simulink model "tractor_mu1109"  (R2022b)
settings: Solver=FixedStepDiscrete  StartTime=0.0  StopTime=20  FixedStep=0.001  RelTol=1e-3
model workspace (MAT data in the model file):
  P : object (value not decoded)
  w_2 : Simulink.Parameter (value not decoded)
undefined symbols (not defined in the file): A, a, B, b, C, D, DiscIntNeverNeededParam, Iz, K, k1, K1, k2, K2, L1, L2, m, magnitude, Phi, Sample_time, Steer_Ratio
libraries: simulink x26, slpidlib x13, Solver_SF x1, dsparch4 x1
(part 3 of 7)

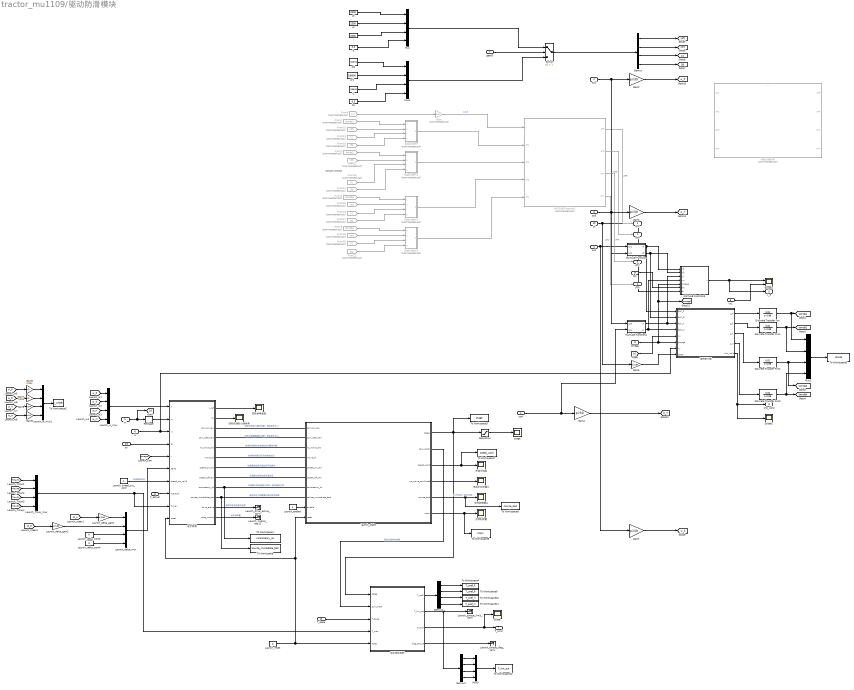
== system tractor_mu1109/驱动防滑模块 ==
  note: 300000
      | 450000
  sp1 : Inport
  sp2 : Inport  Port=2
  sp3 : Inport  Port=3
  sp4 : Inport  Port=4
  vx : Inport  Port=5
  vy : Inport  Port=6
  gearD : Inport  Port=7
  omega : Inport  Port=8
  brk : Inport  Port=9
  st : Inport  Port=10
  T_base : Inport  Port=11
  T_actual : Inport  Port=12
  ax : Inport  Port=13
  Demux : Demux
  Demux1 : Demux
  Demux2 : Demux
  Discrete Transfer Fcn{,1..3} (4 alike) : DiscreteTransferFcn  Numerator=[0.02]  Denominator=[1 -0.98]
  From10 : From  Commented=on  GotoTag=pf
  From{11,13,16,20} (4 alike) : From  Commented=on  GotoTag=i
  From12 : From  Commented=on  GotoTag=pf
  From{14,17..18,21} (4 alike) : From  Commented=on  GotoTag=b
  From15 : From  Commented=on  GotoTag=pr
  From19 : From  Commented=on  GotoTag=pr
  From2 : From  Commented=on  GotoTag=lamda1  TagVisibility=global
  From3 : From  Commented=on  GotoTag=lamda2  TagVisibility=global
  From4 : From  Commented=on  GotoTag=lamda3  TagVisibility=global
  From5 : From  Commented=on  GotoTag=lamda4  TagVisibility=global
  From6 : From  Commented=on  GotoTag=v
  Gain : Gain  Commented=on  Gain=3.6
  Gain{1..4} (4 alike) : Gain  Gain=pi/30
  Gain5 : Gain  Gain=pi/180
  Gain6 : Gain  Gain=0.834
  Gain7 : Gain  Gain=0.834
  Gain8 : Gain  Gain=0.94
  Gain9 : Gain  Gain=0.94
  Launch_Tmax_mux : Mux
  Launch_delta_gain1 : Gain  Gain=pi/180
  Launch_delta_gain2 : Gain  Gain=pi/180
  Launch_delta_mux : Mux
  Launch_delta_zero3 : Constant  Value=0
  Launch_delta_zero4 : Constant  Value=0
  Launch_drive_active_term : Terminator
  Launch_enable : Constant
  Launch_motion_obs12 : Terminator
  Launch_reset : Constant  Value=0
  Launch_speed_src_valid : Constant
  Launch_torque_diag_term : Terminator
  Launch_torque_limit_term : Terminator
  Launch_w_mux : Mux
  Launch_w_mux1 : Mux
  MATLAB Function : MATLAB Function  TreatAsAtomicUnit=on
  MATLAB Function1 : MATLAB Function  TreatAsAtomicUnit=on
  MATLAB Function2 : MATLAB Function  Commented=on  TreatAsAtomicUnit=on
  MATLAB Function3 : MATLAB Function  TreatAsAtomicUnit=on
  Mux{,1..3} (4 alike) : Mux
  Reshape : Reshape  OutputDimensionality=Customize  OutputDimensions=[1 1]
  Saturation : Saturate  UpperLimit=10  LowerLimit=0
  Scope : Scope
  Scope1 : Scope  NumInputPorts=2
  Scope2 : Scope
  Subsystem : Subsystem  Commented=on
  Subsystem1 : Subsystem  Commented=on
  Subsystem2 : Subsystem  Commented=on
  Subsystem3 : Subsystem  Commented=on
  Switch : Switch  Criteria=u2 > Threshold  Threshold=1  SaturateOnIntegerOverflow=off  InputSameDT=off
  To Workspace : ToWorkspace  VariableName=source_immediate_bad  SampleTime=-1
  To Workspace1 : ToWorkspace  VariableName=consistency_ok  SampleTime=-1
  To Workspace10 : ToWorkspace  VariableName=T_pref_rl  SampleTime=-1
      settings: Save2DSignal=2-D array (concatenate along first dimension)
  To Workspace11 : ToWorkspace  VariableName=T_pref_rr  SampleTime=-1
      settings: Save2DSignal=2-D array (concatenate along first dimension)
  To Workspace12 : ToWorkspace  VariableName=T_lim_out  SampleTime=-1
  To Workspace2 : ToWorkspace  VariableName=v_wheel  SampleTime=-1
  To Workspace3 : ToWorkspace  VariableName=stage  SampleTime=-1
  To Workspace4 : ToWorkspace  VariableName=T_pref_fl  SampleTime=-1
      settings: Save2DSignal=2-D array (concatenate along first dimension)
  To Workspace5 : ToWorkspace  VariableName=lamda  SampleTime=-1
  To Workspace6 : ToWorkspace  VariableName=nspin  SampleTime=-1
  To Workspace7 : ToWorkspace  VariableName=speed_valid  SampleTime=-1
  To Workspace8 : ToWorkspace  VariableName=source_bad  SampleTime=-1
  To Workspace9 : ToWorkspace  VariableName=T_pref_fr  SampleTime=-1
      settings: Save2DSignal=2-D array (concatenate along first dimension)
  b : Constant  Value=0.3
  b1 : Constant  Value=0.3
  i : Constant  Value=2000
  i1 : Constant  Value=35000
  launch_state : Stateflow chart  TreatAsAtomicUnit=on
  pf : Constant  Value=2000
  pf1 : Constant  Value=90000
  pr : Constant  Value=2500
  pr1 : Constant  Value=105000
  stage : Scope
  vx1 : InportShadow  Port=5
  信号故障确认 : Scope
  四轮参考速度 : Scope
  四轮轮端轮心速度差 : Scope
  未起步状态确认 : Scope
  滑转率计算 : Subsystem
  空转轮数量 : Scope
  起步扭矩控制 : MATLAB Function  TreatAsAtomicUnit=on
  起步探测 : MATLAB Function  TreatAsAtomicUnit=on
  车速可信度 : Scope
  转矩协调控制 : Stateflow chart  Commented=on  TreatAsAtomicUnit=on
      settings: PortSchema="{\"entries\":[{\"content\":{\"sides\":[{\"content\":{\"connectorIds\":[\"In2\",\"In3\",\"In4\",\"In5\"]},\"type\":\"ConnectorPlacement.EquallySpacedRectSide\",\"uuid\":\"973a9b84-73ad-47b8-a26a-d7aec675acf5\"},{\"content\":{\"connectorIds\":[\"Out1\",\"Out2\",\"Out3\",\"Out4\"],\"side\":\"RIGHT\"},\"type\":\"ConnectorPlacement.EquallySpacedRectSide\",\"uuid\":\"de1e0d9b-25bd-4ac7-be2f-c0268a60ba4f\"},{\"content\":{\"connectorIds\":[\"In1\"],\"side\":\"TOP\"},\"type\":\"ConnectorPlacement.EquallySpacedRectSide\",\"uuid\":\"9ce864d3-2ff1-442a-967b-03df7267dcea\"}]},\"type\":\"ConnectorPlacement.EquallySpacedConnector\",\"uuid\":\"50a94803-c5b1-4606-ba3c-9c5c7d907f69\"}],\"packageUris\":[\"http://schema.mathworks.com/mf0/Connector/R2020b\"],\"version\":\"1.0\"}"
  dTfl : Outport
  dTfr : Outport  Port=2
  dTrl : Outport  Port=3
  dTrr : Outport  Port=4
  v_e : Outport  Port=5
  slip_valid : Outport  Port=6
  T_cmd : Outport  Port=7
  tag scope: lamda1=global, lamda2=global, lamda3=global, lamda4=global, w_fl=global, w_fr=global, w_rl=global, w_rr=global
  wires:
  [w_fl] -> Launch_w_mux/1
  pf/1 -> Mux/1
  pr/1 -> Mux/2
  i/1 -> Mux/3
  [st_R] -> Launch_delta_gain2/1
  b/1 -> Mux/4
  [TMaxRL] -> Launch_Tmax_mux/3
  pf1/1 -> Mux1/1
  pr1/1 -> Mux1/2
  Mux1/1 -> Switch/3
  Subsystem/1(dT1) -> MATLAB Function2/2(dT1)
  i1/1 -> Mux1/3
  b1/1 -> Mux1/4
  launch_state/6(nspin) -> To Workspace6/1, 空转轮数量/1
  From6/1 -> Gain/1
  From2/1 -> Subsystem/1(lamda1)
  From10/1 -> Subsystem/2(p)
  Subsystem3/1(dT1) -> MATLAB Function2/5(dT4)
  From11/1 -> Subsystem/3(i)
  [w_fr] -> Launch_w_mux/2
  From18/1 -> Subsystem/4(b)
  Launch_Tmax_mux/1 -> 起步探测/9(T_max), 起步扭矩控制/4(T_max)
  From4/1 -> Subsystem2/1(lamda3)
  From3/1 -> Subsystem1/1(lamda2)
  From12/1 -> Subsystem1/2(p)
  From14/1 -> Subsystem1/4(b)
  From13/1 -> Subsystem1/3(i)
  sp1/1 -> MATLAB Function/1(sp1), Gain1/1
  From15/1 -> Subsystem2/2(p)
  MATLAB Function2/4(dTrr) -> dTrr/1  "dTrr"
  From16/1 -> Subsystem2/3(i)
  起步扭矩控制/2(T_lim_out) -> Demux2/1, Launch_torque_limit_term/1
  Launch_enable/1 -> launch_state/9(enable)
  From17/1 -> Subsystem2/4(b)
  From5/1 -> Subsystem3/1(lamda4)
  From21/1 -> Subsystem3/4(b)
  From19/1 -> Subsystem3/2(p)
  [st_L] -> Launch_delta_gain1/1
  From20/1 -> Subsystem3/3(i)
  Launch_reset/1 -> 起步扭矩控制/5(reset), launch_state/10(reset), 起步探测/10(reset)
  [TMaxFL] -> Launch_Tmax_mux/1
  st/1 -> MATLAB Function3/7(st), Gain5/1
  [TMaxFR] -> Launch_Tmax_mux/2
  [TMaxRR] -> Launch_Tmax_mux/4
  Mux/1 -> Switch/1
  gearD/1 -> Switch/2
  MATLAB Function2/1(dTfl) -> dTfl/1  "dTfl"
  Launch_w_mux/1 -> 起步探测/1(w)
  launch_state/1(stage) -> To Workspace3/1, Saturation/1, 起步扭矩控制/1(stage)  "工作状态（起步过程）"
  Gain/1 -> MATLAB Function2/1(v)  "km/h"
  Subsystem1/1(dT1) -> MATLAB Function2/3(dT2)
  [w_rl] -> Launch_w_mux/3
  launch_state/2(spin_mask) -> 起步扭矩控制/2(spin_mask)  "四轮空转锁存结果"
  Subsystem2/1(dT1) -> MATLAB Function2/4(dT3)
  launch_state/3(speed_valid) -> To Workspace7/1, 车速可信度/1
  launch_state/4(no_move_confirmed) -> 未起步状态确认/1
  launch_state/5(source_bad) -> To Workspace8/1, 信号故障确认/1
  T_base/1 -> 起步扭矩控制/3(T_base)
  Switch/1 -> Demux/1
  sp2/1 -> MATLAB Function/2(sp2), Gain2/1
  MATLAB Function2/2(dTfr) -> dTfr/1  "dTfr"
  MATLAB Function2/3(dTrl) -> dTrl/1  "dTrl"
  ax/1 -> 起步探测/4(ax)
  sp3/1 -> MATLAB Function1/1(sp3), Gain3/1
  Gain2/1 -> [w_fr]
  起步扭矩控制/3(T_cmd) -> Scope/1, T_cmd/1
  起步扭矩控制/4(diag_torque) -> Launch_torque_diag_term/1
  sp4/1 -> MATLAB Function1/2(sp4), Gain4/1
  [w_rr] -> Launch_w_mux/4
  Launch_delta_gain1/1 -> Launch_delta_mux/1
  Launch_delta_gain2/1 -> Launch_delta_mux/2
  Launch_delta_zero3/1 -> Launch_delta_mux/3
  Launch_delta_zero4/1 -> Launch_delta_mux/4
  Demux/1 -> [pf]
  Demux/2 -> [pr]
  滑转率计算/4(s_rr) -> Discrete Transfer Fcn3/1
  Demux/3 -> [i]
  Demux/4 -> [b]
  Gain3/1 -> [w_rl]
  MATLAB Function/1(vfl) -> MATLAB Function3/1(vfl), 滑转率计算/1(Roll_fl)
  MATLAB Function/2(vfr) -> MATLAB Function3/2(vfr), 滑转率计算/2(Roll_fr)
  brk/1 -> MATLAB Function3/6(brk)
  MATLAB Function1/1(vrl) -> MATLAB Function3/3(vrl), 滑转率计算/3(Roll_rl)
  MATLAB Function1/2(vrr) -> MATLAB Function3/4(vrr), 滑转率计算/4(Roll_rr)
  omega/1 -> [omega], MATLAB Function3/5(omega), 滑转率计算/6(omega)
  [v] -> 滑转率计算/5(vx)
  Gain5/1 -> 滑转率计算/8(derta)
  vy/1 -> 滑转率计算/7(vy), 起步探测/3(vy)
  vx/1 -> [v], Reshape/1
  Gain1/1 -> [w_fl]
  [omega] -> 起步探测/5(r)
  Launch_delta_mux/1 -> 起步探测/6(delta)
  Launch_speed_src_valid/1 -> 起步探测/7(speed_src_valid)  "车速源有效性"
  Gain4/1 -> [w_rr]
  MATLAB Function3/1(v) -> Scope1/1, v_e/1
  vx1/1 -> Scope1/2
  滑转率计算/1(s_fl) -> Discrete Transfer Fcn/1
  滑转率计算/2(s_fr) -> Discrete Transfer Fcn1/1
  滑转率计算/3(s_rl) -> Discrete Transfer Fcn2/1
  滑转率计算/5(slip_valid) -> slip_valid/1, Scope2/1
  起步探测/1(v_ref) -> 四轮参考速度/1
  起步探测/2(dv) -> 四轮轮端轮心速度差/1
  起步探测/3(spin_on_raw) -> launch_state/1(spin_on_raw)  "四轮空转进入瞬时判据，满足条件为 1"
  起步探测/4(spin_clear_raw) -> launch_state/2(spin_clear_raw)  "四轮空转解除瞬时判据，满足条件为 1"
  起步探测/5(no_move_raw) -> launch_state/3(no_move_raw)  "检测到车辆仍未有效起步的瞬时判据"
  起步探测/6(move_ok) -> launch_state/4(move_ok)  "检测到车辆已经开始有效运动"
  起步探测/7(speed_on_raw) -> launch_state/5(speed_on_raw)  "车速源有效且车速达到可信条件"
  起步探测/8(speed_off_raw) -> launch_state/6(speed_off_raw)  "车速源立即失效或车速过低"
  起步探测/9(consistency_ok) -> To Workspace1/1, launch_state/7(consistency_ok)  "车速微分和加速度之间的一致性是否正常"
  起步探测/10(source_immediate_bad) -> To Workspace/1, launch_state/8(source_immediate_bad)  "是否存在立即需要处理的信号故障"
  起步探测/11(drive_active) -> Launch_drive_active_term/1  "是否存在有效驱动扭矩"
  起步探测/12(diag_motion) -> Launch_motion_obs12/1  "运动诊断量"
  Discrete Transfer Fcn/1 -> Mux2/1, [lamda1]
  Discrete Transfer Fcn1/1 -> Mux2/2, [lamda2]
  Discrete Transfer Fcn2/1 -> Mux2/3, [lamda3]
  Discrete Transfer Fcn3/1 -> Mux2/4, [lamda4]
  Reshape/1 -> 起步探测/2(vx)
  Saturation/1 -> stage/1
  T_actual/1 -> 起步探测/8(T_actual)
  [w_fl] -> Gain6/1
  [w_fr] -> Gain7/1
  [w_rl] -> Gain8/1
  [w_rr] -> Gain9/1
  Gain6/1 -> Launch_w_mux1/1
  Gain7/1 -> Launch_w_mux1/2
  Gain8/1 -> Launch_w_mux1/3
  Gain9/1 -> Launch_w_mux1/4
  Launch_w_mux1/1 -> To Workspace2/1
  Mux2/1 -> To Workspace5/1
  起步扭矩控制/1(T_pref) -> Demux1/1
  Demux1/1 -> To Workspace4/1
  Demux1/2 -> To Workspace9/1
  Demux1/3 -> To Workspace10/1
  Demux1/4 -> To Workspace11/1
  Demux2/1 -> Mux3/1
  Demux2/2 -> Mux3/2
  Demux2/3 -> Mux3/3
  Demux2/4 -> Mux3/4
  Mux3/1 -> To Workspace12/1

== system tractor_mu1109/Dugoff轮胎模型/alpha_lamda ==
  vx : Inport
  vy : Inport  Port=2
  wz : Inport  Port=3
  delta_fl : Inport  Port=4
  delta_fr : Inport  Port=5
  w_fl : Inport  Port=6
  w_fr : Inport  Port=7
  w_rl : Inport  Port=8
  w_rr : Inport  Port=9
  Scope : Scope  NumInputPorts=4
  alpha : Subsystem
  lamda : Subsystem
  lamda_fl : Outport
  lamda_fr : Outport  Port=2
  lamda_rl : Outport  Port=3
  lamda_rr : Outport  Port=4
  alpha_fl : Outport  Port=5
  alpha_fr : Outport  Port=6
  alpha_rl : Outport  Port=7
  alpha_rr : Outport  Port=8
  wires:
  lamda/3(lamda_rl) -> Scope/3, lamda_rl/1
  lamda/4(lamda_rr) -> Scope/4, lamda_rr/1
  lamda/2(lamda_fr) -> Scope/2, lamda_fr/1
  lamda/1(lamda_fl) -> Scope/1, lamda_fl/1
  w_rr/1 -> lamda/9(w_rr)
  w_rl/1 -> lamda/8(w_rl)
  w_fr/1 -> lamda/7(w_fr)
  w_fl/1 -> lamda/6(w_fl)
  delta_fr/1 -> alpha/5(delta_fr), lamda/5(delta_fr)
  delta_fl/1 -> alpha/4(delta_fl), lamda/4(delta_fl)
  wz/1 -> alpha/3(wz), lamda/3(wz)
  vy/1 -> alpha/2(vy), lamda/2(vy)
  vx/1 -> alpha/1(vx), lamda/1(vx)
  alpha/4(alpha_rr) -> alpha_rr/1
  alpha/3(alpha_rl) -> alpha_rl/1
  alpha/2(alpha_fr) -> alpha_fr/1
  alpha/1(alpha_fl) -> alpha_fl/1

== system tractor_mu1109/Dugoff轮胎模型/pac2002 ==
  lamda_fl : Inport
  lamda_fr : Inport  Port=2
  lamda_rl : Inport  Port=3
  lamda_rr : Inport  Port=4
  alpha_fl : Inport  Port=5
  alpha_fr : Inport  Port=6
  alpha_rl : Inport  Port=7
  alpha_rr : Inport  Port=8
  Fz_fl : Inport  Port=9
  Fz_rl : Inport  Port=10
  Fz_fr : Inport  Port=11
  Fz_rr : Inport  Port=12
  mu : Inport  Port=13
  Demux : Demux
  Gain{8..11} (4 alike) : Gain  Gain=-1
  fl_dugoff : MATLAB Function  TreatAsAtomicUnit=on
  fr_dugoff : MATLAB Function  TreatAsAtomicUnit=on
  rl_dugoff : MATLAB Function  TreatAsAtomicUnit=on
  rr_dugoff : MATLAB Function  TreatAsAtomicUnit=on
  Fx_fl : Outport
  Fx_fr : Outport  Port=2
  Fx_rl : Outport  Port=3
  Fx_rr : Outport  Port=4
  Fy_fl : Outport  Port=5
  Fy_fr : Outport  Port=6
  Fy_rl : Outport  Port=7
  Fy_rr : Outport  Port=8
  wires:
  alpha_fl/1 -> fl_dugoff/4(alpha)
  Fz_fl/1 -> fl_dugoff/1(Fz)
  alpha_rr/1 -> rr_dugoff/4(alpha)
  Fz_rr/1 -> rr_dugoff/1(Fz)
  [u_fl] -> fl_dugoff/2(u)
  [u_fr] -> fr_dugoff/2(u)
  alpha_fr/1 -> fr_dugoff/4(alpha)
  [u_rl] -> rl_dugoff/2(u)
  [u_rr] -> rr_dugoff/2(u)
  lamda_fr/1 -> Gain11/1
  lamda_rl/1 -> Gain8/1
  lamda_rr/1 -> Gain9/1
  lamda_fl/1 -> Gain10/1
  alpha_rl/1 -> rl_dugoff/4(alpha)
  Gain8/1 -> rl_dugoff/3(lamda)
  Gain9/1 -> rr_dugoff/3(lamda)
  Gain10/1 -> fl_dugoff/3(lamda)
  Gain11/1 -> fr_dugoff/3(lamda)
  mu/1 -> Demux/1
  Demux/1 -> [u_fl]
  Demux/2 -> [u_fr]
  Demux/3 -> [u_rl]
  Demux/4 -> [u_rr]
  Fz_rl/1 -> rl_dugoff/1(Fz)
  Fz_fr/1 -> fr_dugoff/1(Fz)
  fl_dugoff/4(Fy) -> Fy_fl/1
  fl_dugoff/3(Fx) -> Fx_fl/1
  fr_dugoff/4(Fy) -> Fy_fr/1
  fr_dugoff/3(Fx) -> Fx_fr/1
  rl_dugoff/4(Fy) -> Fy_rl/1
  rl_dugoff/3(Fx) -> Fx_rl/1
  rr_dugoff/4(Fy) -> Fy_rr/1
  rr_dugoff/3(Fx) -> Fx_rr/1

== system tractor_mu1109/PID_Controller//直线循迹/Enabled Subsystem ==
  note: DOB:仿真步长Ts=0.001，时间常数Tao=0.1
      | 如需部署到实车需要根据实车采样频率调整
  yaw_ref : Inport
  yaw : Inport  Port=2
  beta : Inport  Port=3
  omega : Inport  Port=4
  Enable : EnablePort  StatesWhenEnabling=reset
  5500/3000 : slpidlib/PID Controller  Controller=PID  Form=Parallel  TimeDomain=Discrete-time  UseExternalTs=off  SampleTime=-1  IntegratorMethod=Forward Euler  FilterMethod=Forward Euler  ControllerParametersSource=internal  P=5500  I=3500  UseKiTs=off  D=0  N=100  UseFilter=on  TunerSelectOption=Transfer Function Based (PID Tuner App)  InitialConditionSource=internal  InitialConditionForIntegrator=0  InitialConditionForFilter=0  DifferentiatorICPrevScaledInput=0  ExternalReset=none  TrackingMode=off  Kt=1  LimitOutput=off  SatLimitsSource=internal  UpperSaturationLimit=inf  LowerSaturationLimit=-inf  LinearizeAsGain=on  AntiWindupMode=none  Kb=1  LimitIntegrator=off  UpperIntegratorSaturationLimit=inf  LowerIntegratorSaturationLimit=-inf  POutMin=[]  POutMax=[]  IOutMin=[]  IOutMax=[]  DOutMin=[]  DOutMax=[]  NOutMin=[]  NOutMax=[]  SumOutMin=[]  SumOutMax=[]  SaturationOutMin=[]  SaturationOutMax=[]  PParamMin=[]  PParamMax=[]  IParamMin=[]  IParamMax=[]  DParamMin=[]  DParamMax=[]  NParamMin=[]  NParamMax=[]  KbParamMin=[]  KbParamMax=[]  KtParamMin=[]  KtParamMax=[]  KbOutMin=[]  KbOutMax=[]  KtOutMin=[]  KtOutMax=[]  IntegratorOutMin=[]  IntegratorOutMax=[]  FilterOutMin=[]  FilterOutMax=[]  SumI1OutMin=[]  SumI1OutMax=[]  SumI2OutMin=[]  SumI2OutMax=[]  SumI3OutMin=[]  SumI3OutMax=[]  SumI4OutMin=[]  SumI4OutMax=[]  SumDOutMin=[]  SumDOutMax=[]  DifferentiatorOutMin=[]  DifferentiatorOutMax=[]  FilterDiffOutCoefMin=[]  FilterDiffOutCoefMax=[]  ReciprocalOutMin=[]  ReciprocalOutMax=[]  SumDenOutMin=[]  SumDenOutMax=[]  SumNumOutMin=[]  SumNumOutMax=[]  DivideOutMin=[]  DivideOutMax=[]  UdiffTsProdOutMin=[]  UdiffTsProdOutMax=[]  NTsProdOutMin=[]  NTsProdOutMax=[]  UintegralTsProdOutMin=[]  UintegralTsProdOutMax=[]  UngainTsProdOutMin=[]  UngainTsProdOutMax=[]  ClampingZeroOutDataTypeStr=Inherit: Inherit via back propagation  ClampingZeroOutMin=[]  ClampingZeroOutMax=[]  FilterDenConstantOutDataTypeStr=Inherit: Inherit via back propagation  FilterDenConstantOutMin=[]  FilterDenConstantOutMax=[]  PCopyOutDataTypeStr=Inherit: Inherit via back propagation  PCopyOutMin=[]  PCopyOutMax=[]  NCopyOutDataTypeStr=Inherit: Inherit via back propagation  NCopyOutMin=[]  NCopyOutMax=[]  IntegratorContinuousStateAttributes=''  IntegratorStateMustResolveToSignalObject=off  IntegratorRTWStateStorageClass=Auto  FilterContinuousStateAttributes=''  FilterStateMustResolveToSignalObject=off  FilterRTWStateStorageClass=Auto  ParallelPVariant=InternalParameters  IdealPVariant=Disabled  IVariant=InternalParameters  DVariant=InternalParameters  IntegratorVariant=Discrete  SatVariant=Disabled  AWVariant=Passthrough  PCopyVariant=Disabled  TRVariant=Disabled  FdbkBlocksVariant=Forward  IdealPFdbkVariant=Disabled  SatFdbkVariant=Disabled  DerivativeFilterVariant=ForwardEulerFilter  NVariant=InternalParameters  NCopyVariant=Disabled  FilterICVariant=InternalICsFilter  IntegratorICVariant=InternalICs  ExternalResetVariant=Disabled  TRSumVariant=Passthrough  SumFdbkVariant=Disabled  SumVariant=Sum_PID  TsampFilterVariant=InternalTs  TsampNgainVariant=Passthrough  TsampIntegralVariant=Passthrough  ExternalSaturationOutDataTypeStr=Inherit: Same as second input
  Add : Sum  Inputs=+++
  Data Type Conversion : DataTypeConversion  OutDataTypeStr=single  SaturateOnIntegerOverflow=off  RndMeth=Floor
  Data Type Conversion1 : DataTypeConversion  OutDataTypeStr=single  SaturateOnIntegerOverflow=off  RndMeth=Floor
  Discrete Transfer Fcn : DiscreteTransferFcn  Numerator=[1-exp(-0.2)]  Denominator=[1 -exp(-0.2)]
  Gain : Gain  Gain=-1
  Gain1 : Gain  Gain=-K(1)
  Gain2 : Gain  Gain=-K(2)
  Gain3 : Gain  Gain=-K(3)
  Gain4 : Gain  Gain=3
  Gain5 : Gain  Gain=0.5
  Gain6 : Gain  Gain=180/pi
  Izr_dot : simulink/Discrete/Discrete Derivative  gainval=67536  ICPrevScaledInput=0.0  OutMin=[]  OutMax=[]  OutDataType=fixdt(1, 16)  OutScaling=2^-10  DoSatur=off
  Manual Switch : ManualSwitch
  Manual Switch1 : ManualSwitch
  Subtract : Sum  Inputs=+-
  Sum : Sum  Inputs=|+-
  Sum2 : Sum  Inputs=|+-
  Mz : Outport
  wires:
  5500/3000/1 -> Data Type Conversion1/1
  yaw_ref/1 -> Sum/1
  yaw/1 -> Sum/2
  Sum/1 -> Gain/1, Gain6/1
  Sum2/1 -> Manual Switch/2
  Discrete Transfer Fcn/1 -> Gain5/1
  Subtract/1 -> Discrete Transfer Fcn/1
  Gain3/1 -> Add/3  "eyaw"
  Gain1/1 -> Add/1  "beta"
  Izr_dot/1 -> Subtract/1
  omega/1 -> Izr_dot/1, Gain2/1
  Gain2/1 -> Add/2  "omega"
  Add/1 -> Gain4/1
  beta/1 -> Gain1/1
  Gain/1 -> Gain3/1
  Manual Switch/1 -> Manual Switch1/2
  Manual Switch1/1 -> Mz/1
  Gain4/1 -> Subtract/2, Manual Switch/1, Sum2/1
  Data Type Conversion/1 -> Sum2/2  "Mz_DOB"
  Data Type Conversion1/1 -> Manual Switch1/1  "Mz_pid"
  Gain5/1 -> Data Type Conversion/1
  Gain6/1 -> 5500/3000/1

== system tractor_mu1109/PID_Controller//直线循迹/目标航向角计算 ==
  reset : Inport
  yaw : Inport  Port=2
  omega : Inport  Port=3
  Enable : EnablePort  StatesWhenEnabling=reset
  Abs : Abs  SaturateOnIntegerOverflow=off
  Add : Sum
  Constant : Constant
  Constant1 : Constant  Value=0.001
  Discrete-Time Integrator : DiscreteIntegrator  ExternalReset=rising  SampleTime=-1  ICPrevOutput=DiscIntNeverNeededParam  ICPrevScaledInput=DiscIntNeverNeededParam
  Discrete-Time Integrator1 : DiscreteIntegrator  ExternalReset=rising  SampleTime=-1  ICPrevOutput=DiscIntNeverNeededParam  ICPrevScaledInput=DiscIntNeverNeededParam
  Divide : Product  Inputs=*/
  Divide1 : Product  Inputs=*/
  Product : Product
  Saturation : Saturate  UpperLimit=999999  LowerLimit=0.1
  yaw_r : Outport
  wires:
  Constant/1 -> Divide/1
  omega/1 -> Abs/1
  Abs/1 -> Add/1
  Constant1/1 -> Add/2
  Add/1 -> Divide/2
  Divide/1 -> Discrete-Time Integrator1/1, Product/2
  yaw/1 -> Product/1
  Product/1 -> Discrete-Time Integrator/1
  Discrete-Time Integrator/1 -> Divide1/1
  Discrete-Time Integrator1/1 -> Saturation/1
  Divide1/1 -> yaw_r/1
  Saturation/1 -> Divide1/2
  reset/1 -> Discrete-Time Integrator1/2, Discrete-Time Integrator/2

== system tractor_mu1109/协同博弈扭矩分配/Subsystem ==
  Tflref : Inport
  Tfrref : Inport  Port=2
  Trlref : Inport  Port=3
  Trrref : Inport  Port=4
  Tflbase : Inport  Port=5
  Tfrbase : Inport  Port=6
  Trlbase : Inport  Port=7
  Trrbase : Inport  Port=8
  alpha : Inport  Port=9
  Constant{,1..3} (4 alike) : Constant
  Product{,1..7} (8 alike) : Product
  Sum{,2,4,6} (4 alike) : Sum  Inputs=|+-
  Sum{1,3,5,7} (4 alike) : Sum  Inputs=|++
  alpha1 : InportShadow  Port=9
  alpha2 : InportShadow  Port=9
  alpha3 : InportShadow  Port=9
  Tfl_sh : Outport
  Tfr_sh : Outport  Port=2
  Trl_sh : Outport  Port=3
  Trr_sh : Outport  Port=4
  wires:
  Tflbase/1 -> Product/1
  Constant/1 -> Sum/1
  alpha/1 -> Sum/2, Product1/2
  Sum/1 -> Product/2
  Product/1 -> Sum1/1
  Product1/1 -> Sum1/2
  Tflref/1 -> Product1/1
  Sum1/1 -> Tfl_sh/1
  Sum3/1 -> Tfr_sh/1
  Tfrref/1 -> Product3/1
  Product3/1 -> Sum3/2
  Product2/1 -> Sum3/1
  Sum2/1 -> Product2/2
  alpha1/1 -> Product3/2, Sum2/2
  Constant1/1 -> Sum2/1
  Tfrbase/1 -> Product2/1
  Trlbase/1 -> Product4/1
  Constant2/1 -> Sum4/1
  alpha2/1 -> Sum4/2, Product5/2
  Sum4/1 -> Product4/2
  Product4/1 -> Sum5/1
  Product5/1 -> Sum5/2
  Trlref/1 -> Product5/1
  Sum5/1 -> Trl_sh/1
  Sum7/1 -> Trr_sh/1
  Trrref/1 -> Product7/1
  Product7/1 -> Sum7/2
  Product6/1 -> Sum7/1
  Sum6/1 -> Product6/2
  alpha3/1 -> Product7/2, Sum6/2
  Constant3/1 -> Sum6/1
  Trrbase/1 -> Product6/1

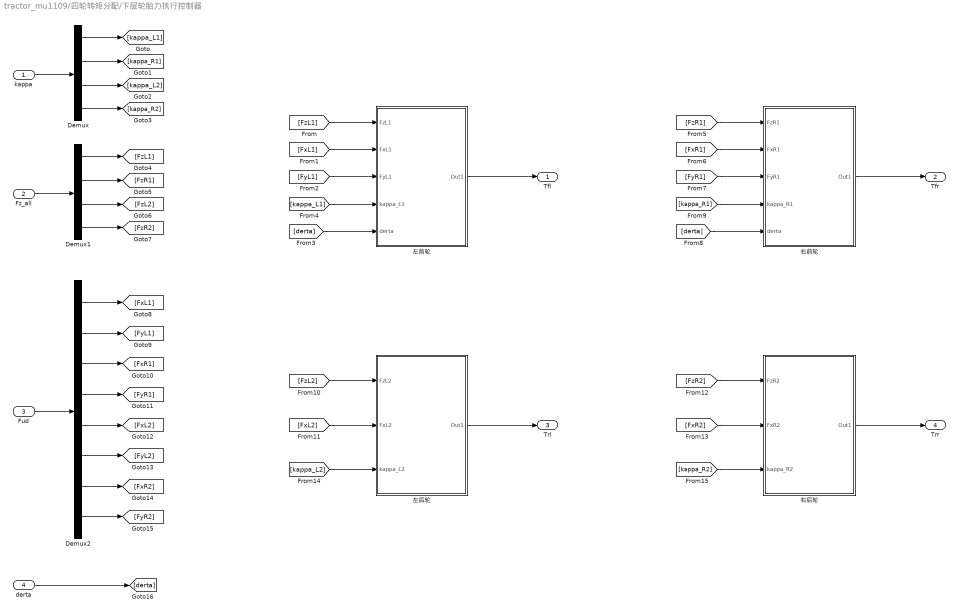
== system tractor_mu1109/四轮转矩分配/下层轮胎力执行控制器 ==
  kappa : Inport
  Fz_all : Inport  Port=2
  Fud : Inport  Port=3
  derta : Inport  Port=4
  Demux : Demux
  Demux1 : Demux
  Demux2 : Demux  Outputs=8
  右前轮 : Subsystem
  右后轮 : Subsystem
  左前轮 : Subsystem
  左后轮 : Subsystem
  Tfl : Outport
  Tfr : Outport  Port=2
  Trl : Outport  Port=3
  Trr : Outport  Port=4
  wires:
  kappa/1 -> Demux/1
  Demux/1 -> [kappa_L1]
  Demux/2 -> [kappa_R1]
  Demux/3 -> [kappa_L2]
  Demux/4 -> [kappa_R2]
  Fz_all/1 -> Demux1/1
  Demux1/1 -> [FzL1]
  Demux1/2 -> [FzR1]
  Demux1/3 -> [FzL2]
  Demux1/4 -> [FzR2]
  Fud/1 -> Demux2/1
  Demux2/1 -> [FxL1]
  Demux2/2 -> [FyL1]
  Demux2/3 -> [FxR1]
  Demux2/4 -> [FyR1]
  Demux2/6 -> [FyL2]
  Demux2/5 -> [FxL2]
  Demux2/8 -> [FyR2]
  Demux2/7 -> [FxR2]
  derta/1 -> [derta]
  左前轮/1(Out1) -> Tfl/1
  [FzL1] -> 左前轮/1(FzL1)
  [FxL1] -> 左前轮/2(FxL1)
  [FyL1] -> 左前轮/3(FyL1)
  [kappa_L1] -> 左前轮/4(kappa_L1)
  [derta] -> 左前轮/5(derta)
  [derta] -> 右前轮/5(derta)
  [kappa_R1] -> 右前轮/4(kappa_R1)
  [FyR1] -> 右前轮/3(FyR1)
  [FxR1] -> 右前轮/2(FxR1)
  [FzR1] -> 右前轮/1(FzR1)
  右前轮/1(Out1) -> Tfr/1
  [kappa_L2] -> 左后轮/3(kappa_L2)
  [FxL2] -> 左后轮/2(FxL2)
  [FzL2] -> 左后轮/1(FzL2)
  左后轮/1(Out1) -> Trl/1
  右后轮/1(Out1) -> Trr/1
  [FzR2] -> 右后轮/1(FzR2)
  [FxR2] -> 右后轮/2(FxR2)
  [kappa_R2] -> 右后轮/3(kappa_R2)

== system tractor_mu1109/总驱动力矩制定/DOB补偿 ==
  note: 仿真时间t=0.001
      | 时间常数tao=0.1
  vx : Inport
  T : Inport  Port=2
  Discrete Transfer Fcn : DiscreteTransferFcn  Numerator=[1 1]  Denominator=[201 -199]
  Discrete Derivative : simulink/Discrete/Discrete Derivative  gainval=1.0  ICPrevScaledInput=0.0  OutMin=[]  OutMax=[]  OutDataType=fixdt(1, 16)  OutScaling=2^-10  DoSatur=off
  Sum : Sum  Inputs=|-+
  m*Rf : Gain  Gain=18530*0.834
  低通LPF : DiscreteTransferFcn  Numerator=[1-0.9802]  Denominator=[1 -0.9802]
  Td_hat : Outport
  wires:
  Discrete Derivative/1 -> m*Rf/1
  vx/1 -> 低通LPF/1
  m*Rf/1 -> Sum/1
  T/1 -> Sum/2
  Sum/1 -> Discrete Transfer Fcn/1
  Discrete Transfer Fcn/1 -> Td_hat/1
  低通LPF/1 -> Discrete Derivative/1

== system tractor_mu1109/总驱动力矩制定/正常工况_高速衰减防抖 ==
  gearD : Inport
  vx : Inport  Port=2
  T0 : Inport  Port=3
  1档 : Switch  Criteria=u2 > Threshold  Threshold=14/3.6  SaturateOnIntegerOverflow=off  InputSameDT=off
  2档 : Switch  Criteria=u2 > Threshold  Threshold=40  SaturateOnIntegerOverflow=off  InputSameDT=off
  Gain14 : Gain  Gain=3.6
  Subsystem1 : Subsystem
  Switch5 : Switch  Criteria=u2 > Threshold  Threshold=1  SaturateOnIntegerOverflow=off  InputSameDT=off
  高速衰减冻结区 : Subsystem
  T : Outport
  wires:
  vx/1 -> 1档/2, Gain14/1
  Gain14/1 -> Subsystem1/1(v), 2档/2, 高速衰减冻结区/1(v)
  T0/1 -> 2档/3, 1档/3
  1档/1 -> Switch5/3
  Subsystem1/1(Out1) -> 2档/1
  高速衰减冻结区/1(Out1) -> 1档/1
  gearD/1 -> Switch5/2
  2档/1 -> Switch5/1
  Switch5/1 -> T/1

== system tractor_mu1109/牵引效率计算/Subsystem1 ==
  T : Inport
  F_hat : Inport  Port=2
  wij : Inport  Port=3
  Fz : Inport  Port=4
  Add : Sum  Inputs=+++-
  Gain : Gain  Gain=50
  Jw : Gain  Gain=1/356.42
  Product : Product
  Saturation : Saturate  UpperLimit=1  LowerLimit=-1
  Sum : Sum  Inputs=|+-
  边界层厚度 : Gain  Gain=1/1
  Fx_out : Outport
  wires:
  wij/1 -> Sum/1
  Sum/1 -> Gain/1, 边界层厚度/1
  边界层厚度/1 -> Saturation/1
  Saturation/1 -> Product/2  "us"
  T/1 -> Jw/1
  Jw/1 -> Add/1
  Gain/1 -> Add/2
  Product/1 -> Add/3

== system tractor_mu1109/牵引效率计算/总纵向力估计 ==
  ax : Inport
  theta : Inport  Port=2
  EFsum : Inport  Port=3
  vx : Inport  Port=4
  Fz4 : Inport  Port=5
  Add : Sum  Inputs=---+
  Add1 : Sum  Inputs=++++
  Delay : Delay  DelayLength=1
  Demux : Demux
  Gain1 : Gain  Gain=2.4516
  Gain3 : Gain  Gain=18530*9.8
  Gain5 : Gain  Gain=18530
  Math Function : Math  Operator=magnitude^2
  Saturation : Saturate  UpperLimit=999999999  LowerLimit=0
  Saturation1 : Saturate  UpperLimit=999999999  LowerLimit=0
  Saturation2 : Saturate  UpperLimit=999999999  LowerLimit=0
  Sin1 : Trigonometry
  Sum : Sum  Inputs=|+-
  Switch : Switch  Criteria=u2 > Threshold  Threshold=0.5  SaturateOnIntegerOverflow=off  InputSameDT=off
  滚动阻力系数 : Gain  Gain=0.02
  R_load : Outport
  R_all : Outport  Port=2
  R_g : Outport  Port=3
  R_f : Outport  Port=4
  R_a : Outport  Port=5
  wires:
  ax/1 -> Gain5/1
  theta/1 -> Sin1/1
  Gain1/1 -> R_a/1, Add/2
  Sin1/1 -> Gain3/1
  Gain3/1 -> R_g/1, Add/3
  Add/1 -> Saturation/1
  EFsum/1 -> Sum/1
  Gain5/1 -> Sum/2
  Sum/1 -> Delay/1, Add/4, Saturation1/1
  Fz4/1 -> Demux/1
  Demux/1 -> Add1/1
  Demux/2 -> Add1/2
  Demux/3 -> Add1/3
  Demux/4 -> Add1/4
  Add1/1 -> 滚动阻力系数/1
  滚动阻力系数/1 -> Add/1, R_f/1
  vx/1 -> Switch/2, Math Function/1
  Math Function/1 -> Gain1/1
  Saturation/1 -> R_load/1
  Saturation1/1 -> Switch/1
  Switch/1 -> R_all/1
  Delay/1 -> Saturation2/1
  Saturation2/1 -> Switch/3

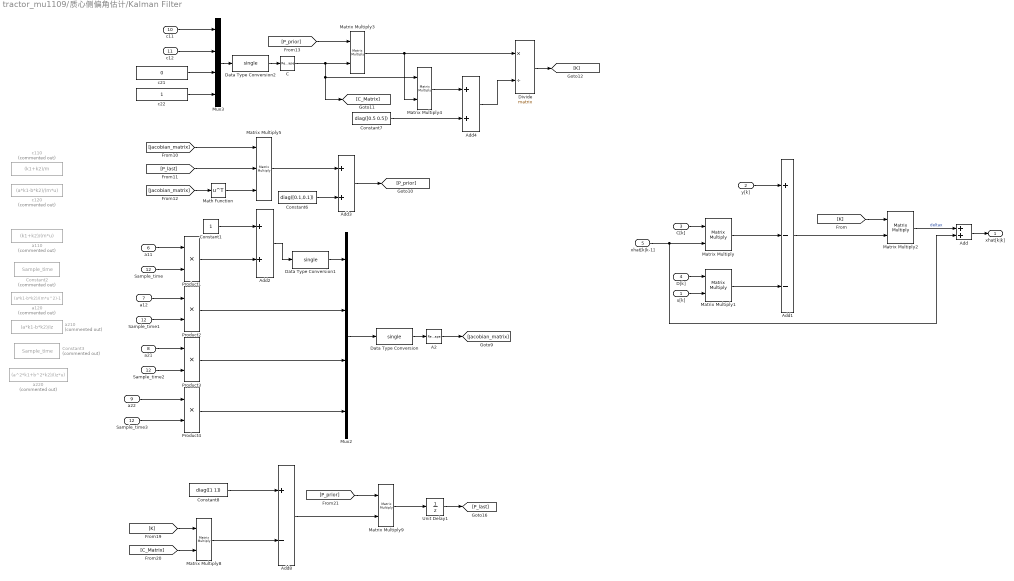
== system tractor_mu1109/质心侧偏角估计/Kalman Filter ==
  u[k] : Inport
  y[k] : Inport  Port=2
  C[k] : Inport  Port=3
  D[k] : Inport  Port=4
  xhat[k|k-1] : Inport  Port=5
  a11 : Inport  Port=6  OutDataTypeStr=single
  a12 : Inport  Port=7  OutDataTypeStr=single
  a21 : Inport  Port=8  OutDataTypeStr=single
  a22 : Inport  Port=9  OutDataTypeStr=single
  c11 : Inport  Port=10  OutDataTypeStr=single
  c12 : Inport  Port=11  OutDataTypeStr=single
  Sample_time : Inport  Port=12  OutDataTypeStr=single
  A2 : Reshape  OutputDimensionality=Customize  OutputDimensions=[2,2]
  Add{,2..4} (4 alike) : Sum
  Add1 : Sum  Inputs=+--
  Add8 : Sum  Inputs=+-
  C : Reshape  OutputDimensionality=Customize  OutputDimensions=[2,2]
  Constant1 : Constant
  Constant2 : Constant  Commented=on  Value=Sample_time
  Constant3 : Constant  Commented=on  Value=Sample_time
  Constant6 : Constant  Value=diag([0.1,0.1])
  Constant7 : Constant  Value=diag([0.5 0.5])
  Constant8 : Constant  Value=diag([1 1])
  Data Type Conversion : DataTypeConversion  OutDataTypeStr=single  SaturateOnIntegerOverflow=off  RndMeth=Floor
  Data Type Conversion1 : DataTypeConversion  OutDataTypeStr=single  SaturateOnIntegerOverflow=off  RndMeth=Floor
  Data Type Conversion2 : DataTypeConversion  OutDataTypeStr=single  SaturateOnIntegerOverflow=off  RndMeth=Floor
  Divide : Product  Inputs=*/  Multiplication=Matrix(*)
  Math Function : Math  Operator=transpose  SignedPower=on
  Matrix Multiply{,1..4,8..9} (7 alike) : Product  Multiplication=Matrix(*)
  Matrix Multiply5 : Product  Inputs=3  Multiplication=Matrix(*)
  Mux2 : Mux
  Mux3 : Mux
  Product1 : Product
  Product2 : Product
  Product3 : Product  OutDataTypeStr=single
  Product4 : Product  OutDataTypeStr=single
  Sample_time1 : InportShadow  Port=12  OutDataTypeStr=single
  Sample_time2 : InportShadow  Port=12  OutDataTypeStr=single
  Sample_time3 : InportShadow  Port=12  OutDataTypeStr=single
  Unit Delay1 : UnitDelay  SampleTime=-1  HasFrameUpgradeWarning=on
  a110 : Constant  Commented=on  Value=(k1+k2)/(m*u)
  a120 : Constant  Commented=on  Value=(a*k1-b*k2)/(m*u^2)-1
  a210 : Constant  Commented=on  Value=(a*k1-b*k2)/Iz
  a220 : Constant  Commented=on  Value=(a^2*k1+b^2*k2)/(Iz*u)
  c110 : Constant  Commented=on  Value=(k1+k2)/m
  c120 : Constant  Commented=on  Value=(a*k1-b*k2)/(m*u)
  c21 : Constant  Value=0  OutDataTypeStr=single
  c22 : Constant  OutDataTypeStr=single
  xhat[k|k] : Outport
  wires:
  Add/1 -> xhat[k|k]/1
  C[k]/1 -> Matrix Multiply/1
  xhat[k|k-1]/1 -> Matrix Multiply/2, Add/2
  D[k]/1 -> Matrix Multiply1/1
  u[k]/1 -> Matrix Multiply1/2
  y[k]/1 -> Add1/1
  Matrix Multiply/1 -> Add1/2
  Matrix Multiply1/1 -> Add1/3
  Add1/1 -> Matrix Multiply2/2
  Matrix Multiply2/1 -> Add/1  "deltax"
  Add4/1 -> Divide/2
  Matrix Multiply3/1 -> Divide/1, Matrix Multiply4/2
  c21/1 -> Mux3/3
  Matrix Multiply4/1 -> Add4/1
  c22/1 -> Mux3/4
  Mux3/1 -> Data Type Conversion2/1
  Constant7/1 -> Add4/2
  c11/1 -> Mux3/1
  [P_prior] -> Matrix Multiply3/1
  C/1 -> Matrix Multiply4/1, [C_Matrix], Matrix Multiply3/2
  Divide/1 -> [K]
  [P_last] -> Matrix Multiply5/2
  Matrix Multiply5/1 -> Add3/1
  [Jacobian_matrix] -> Math Function/1
  Math Function/1 -> Matrix Multiply5/3
  Add3/1 -> [P_prior]
  [Jacobian_matrix] -> Matrix Multiply5/1
  Constant6/1 -> Add3/2
  Sample_time2/1 -> Product3/2
  Sample_time3/1 -> Product4/2
  a12/1 -> Product2/1
  A2/1 -> [Jacobian_matrix]
  Add2/1 -> Data Type Conversion1/1
  Product1/1 -> Add2/2
  Sample_time1/1 -> Product2/2
  a22/1 -> Product4/1
  Mux2/1 -> Data Type Conversion/1
  a21/1 -> Product3/1
  Constant1/1 -> Add2/1
  [K] -> Matrix Multiply2/1
  Matrix Multiply8/1 -> Add8/2
  Constant8/1 -> Add8/1
  Unit Delay1/1 -> [P_last]
  [P_prior] -> Matrix Multiply9/1
  Add8/1 -> Matrix Multiply9/2
  Matrix Multiply9/1 -> Unit Delay1/1
  [K] -> Matrix Multiply8/1
  [C_Matrix] -> Matrix Multiply8/2
  a11/1 -> Product1/1
  c12/1 -> Mux3/2
  Sample_time/1 -> Product1/2
  Product2/1 -> Mux2/2
  Product3/1 -> Mux2/3
  Product4/1 -> Mux2/4
  Data Type Conversion/1 -> A2/1
  Data Type Conversion1/1 -> Mux2/1
  Data Type Conversion2/1 -> C/1

== system tractor_mu1109/质心侧偏角估计/Observer ==
  note: A*xhat+B*u+L*(yMeas-yHat)
      | or
      | A*xhat+B*u
  u[k] : Inport
  y[k] : Inport  Port=2
  A[k] : Inport  Port=3
  B[k] : Inport  Port=4
  C[k] : Inport  Port=5
  D[k] : Inport  Port=6
  L[k] : Inport  Port=7
  xhat[k|k-1] : Inport  Port=8
  Add : Sum  Inputs=+++
  Matrix Multiply : Product  Multiplication=Matrix(*)
  Matrix Multiply1 : Product  Multiplication=Matrix(*)
  Reshape : Reshape
  Subsystem : Subsystem
  x[k+1|k] : Outport
  wires:
  B[k]/1 -> Matrix Multiply/1
  u[k]/1 -> Subsystem/6(u[k]), Matrix Multiply/2
  A[k]/1 -> Matrix Multiply1/1
  xhat[k|k-1]/1 -> Matrix Multiply1/2, Subsystem/4(xhat[k|k-1])
  L[k]/1 -> Subsystem/1(L[k])
  y[k]/1 -> Subsystem/2(y[k])
  C[k]/1 -> Subsystem/3(C[k])
  D[k]/1 -> Subsystem/5(D[k])
  Matrix Multiply/1 -> Add/1
  Matrix Multiply1/1 -> Add/2
  Subsystem/1(L*(y[k]-yhat[k|k-1])) -> Add/3
  Add/1 -> Reshape/1
  Reshape/1 -> x[k+1|k]/1

== system tractor_mu1109/质心侧偏角滑模观测器估计/Subsystem ==
  Avz_Carsim : Inport
  vx : Inport  Port=2
  delta_f : Inport  Port=3
  Atan : Trigonometry  Operator=atan
  Constant : Constant  Value=0.1
  Divide : Product  Inputs=*/
  Gain1 : Gain  Gain=L1
  Gain2 : Gain  Gain=L2
  MATLAB Function : MATLAB Function  TreatAsAtomicUnit=on  SystemSampleTime=0.005
  Scope1 : Scope
  Scope2 : Scope
  Subsystem : Subsystem
  Sum : Sum  Inputs=|+-
  Sum1 : Sum  Inputs=|++
  Sum2 : Sum  Inputs=|++
  Switch : Switch  Criteria=u2 > Threshold  Threshold=0.1  SaturateOnIntegerOverflow=off  InputSameDT=off
  gamma_hat : DiscreteIntegrator  SampleTime=-1  ICPrevOutput=DiscIntNeverNeededParam  ICPrevScaledInput=DiscIntNeverNeededParam
  vy_hat : DiscreteIntegrator  SampleTime=-1  ICPrevOutput=DiscIntNeverNeededParam  ICPrevScaledInput=DiscIntNeverNeededParam
  beta_est : Outport
  gamma_est : Outport  Port=2
  vy_hat_output : Outport  Port=3
  wires:
  Avz_Carsim/1 -> Sum/1
  Sum/1 -> Subsystem/1(error)
  MATLAB Function/1(d_vy_model) -> Sum1/2
  gamma_hat/1 -> Scope1/1, MATLAB Function/4(gamma_hat), gamma_est/1, Sum/2
  vx/1 -> Scope2/1, Switch/1, Switch/2
  Constant/1 -> Switch/3
  vy_hat/1 -> vy_hat_output/1, Divide/1, MATLAB Function/3(vy_hat)
  Switch/1 -> Divide/2, MATLAB Function/1(vx)
  Subsystem/1(v_STA) -> Gain2/1, Gain1/1
  delta_f/1 -> MATLAB Function/2(delta_f)
  Divide/1 -> Atan/1
  Gain1/1 -> Sum1/1
  Gain2/1 -> Sum2/1
  MATLAB Function/2(d_gamma_model) -> Sum2/2
  Atan/1 -> beta_est/1
  Sum1/1 -> vy_hat/1
  Sum2/1 -> gamma_hat/1

== system tractor_mu1109/质心侧偏角滑模观测器估计/Subsystem1 ==
  Avz_Carsim : Inport
  vx : Inport  Port=2
  delta_f : Inport  Port=3
  Atan : Trigonometry  Operator=atan
  Constant : Constant  Value=0.1
  Divide : Product  Inputs=*/
  Gain : Gain  Gain=1/Phi
  Gain1 : Gain  Gain=L1
  Gain2 : Gain  Gain=L2
  MATLAB Function : MATLAB Function  TreatAsAtomicUnit=on  SystemSampleTime=0.005
  Saturation : Saturate  UpperLimit=1  LowerLimit=-1
  Scope1 : Scope
  Scope2 : Scope
  Sum : Sum  Inputs=|+-
  Sum1 : Sum  Inputs=|++
  Sum2 : Sum  Inputs=|++
  Switch : Switch  Criteria=u2 > Threshold  Threshold=0.1  SaturateOnIntegerOverflow=off  InputSameDT=off
  gamma_hat : Integrator
  vy_hat : Integrator
  beta_est : Outport
  gamma_est : Outport  Port=2
  vy_hat_output : Outport  Port=3
  wires:
  Gain/1 -> Saturation/1
  Avz_Carsim/1 -> Sum/1
  Sum/1 -> Gain/1
  MATLAB Function/1(d_vy_model) -> Sum1/2
  gamma_hat/1 -> Scope1/1, MATLAB Function/4(gamma_hat), gamma_est/1, Sum/2
  vx/1 -> Scope2/1, Switch/1, Switch/2
  Constant/1 -> Switch/3
  vy_hat/1 -> vy_hat_output/1, Divide/1, MATLAB Function/3(vy_hat)
  Switch/1 -> Divide/2, MATLAB Function/1(vx)
  Saturation/1 -> Gain2/1, Gain1/1
  delta_f/1 -> MATLAB Function/2(delta_f)
  Divide/1 -> Atan/1
  Gain1/1 -> Sum1/1
  Gain2/1 -> Sum2/1
  MATLAB Function/2(d_gamma_model) -> Sum2/2
  Atan/1 -> beta_est/1
  Sum1/1 -> vy_hat/1
  Sum2/1 -> gamma_hat/1

== system tractor_mu1109/驱动防滑模块/Subsystem ==
  lamda1 : Inport
  p : Inport  Port=2
  i : Inport  Port=3
  b : Inport  Port=4
  Constant : Constant  Value=0.2
  PID Controller : slpidlib/PID Controller  Controller=PI  Form=Parallel  TimeDomain=Discrete-time  UseExternalTs=off  SampleTime=-1  IntegratorMethod=Forward Euler  FilterMethod=Forward Euler  ControllerParametersSource=external  P=5000  I=3000  UseKiTs=off  D=0  N=100  UseFilter=on  TunerSelectOption=Transfer Function Based (PID Tuner App)  InitialConditionSource=internal  InitialConditionForIntegrator=0  InitialConditionForFilter=0  DifferentiatorICPrevScaledInput=0  ExternalReset=none  TrackingMode=off  Kt=1  LimitOutput=on  SatLimitsSource=internal  UpperSaturationLimit=0  LowerSaturationLimit=-30000  LinearizeAsGain=on  AntiWindupMode=clamping  Kb=1  LimitIntegrator=off  UpperIntegratorSaturationLimit=inf  LowerIntegratorSaturationLimit=-inf  POutMin=[]  POutMax=[]  IOutMin=[]  IOutMax=[]  DOutMin=[]  DOutMax=[]  NOutMin=[]  NOutMax=[]  SumOutMin=[]  SumOutMax=[]  SaturationOutMin=[]  SaturationOutMax=[]  PParamMin=[]  PParamMax=[]  IParamMin=[]  IParamMax=[]  DParamMin=[]  DParamMax=[]  NParamMin=[]  NParamMax=[]  KbParamMin=[]  KbParamMax=[]  KtParamMin=[]  KtParamMax=[]  KbOutMin=[]  KbOutMax=[]  KtOutMin=[]  KtOutMax=[]  IntegratorOutMin=[]  IntegratorOutMax=[]  FilterOutMin=[]  FilterOutMax=[]  SumI1OutMin=[]  SumI1OutMax=[]  SumI2OutMin=[]  SumI2OutMax=[]  SumI3OutMin=[]  SumI3OutMax=[]  SumI4OutMin=[]  SumI4OutMax=[]  SumDOutMin=[]  SumDOutMax=[]  DifferentiatorOutMin=[]  DifferentiatorOutMax=[]  FilterDiffOutCoefMin=[]  FilterDiffOutCoefMax=[]  ReciprocalOutMin=[]  ReciprocalOutMax=[]  SumDenOutMin=[]  SumDenOutMax=[]  SumNumOutMin=[]  SumNumOutMax=[]  DivideOutMin=[]  DivideOutMax=[]  UdiffTsProdOutMin=[]  UdiffTsProdOutMax=[]  NTsProdOutMin=[]  NTsProdOutMax=[]  UintegralTsProdOutMin=[]  UintegralTsProdOutMax=[]  UngainTsProdOutMin=[]  UngainTsProdOutMax=[]  ClampingZeroOutDataTypeStr=Inherit: Inherit via back propagation  ClampingZeroOutMin=[]  ClampingZeroOutMax=[]  FilterDenConstantOutDataTypeStr=Inherit: Inherit via back propagation  FilterDenConstantOutMin=[]  FilterDenConstantOutMax=[]  PCopyOutDataTypeStr=Inherit: Inherit via back propagation  PCopyOutMin=[]  PCopyOutMax=[]  NCopyOutDataTypeStr=Inherit: Inherit via back propagation  NCopyOutMin=[]  NCopyOutMax=[]  IntegratorContinuousStateAttributes=''  IntegratorStateMustResolveToSignalObject=off  IntegratorRTWStateStorageClass=Auto  FilterContinuousStateAttributes=''  FilterStateMustResolveToSignalObject=off  FilterRTWStateStorageClass=Auto  ParallelPVariant=ExternalParameters  IdealPVariant=Disabled  IVariant=ExternalParameters  DVariant=Disabled  IntegratorVariant=Discrete  SatVariant=Enabled  AWVariant=DiscClampingParallel  PCopyVariant=Disabled  TRVariant=Disabled  FdbkBlocksVariant=Forward  IdealPFdbkVariant=Disabled  SatFdbkVariant=Disabled  DerivativeFilterVariant=Disabled  NVariant=Disabled  NCopyVariant=Disabled_SignalSpec  FilterICVariant=Disabled  IntegratorICVariant=InternalICs  ExternalResetVariant=Disabled  TRSumVariant=Passthrough  SumFdbkVariant=Disabled  SumVariant=Sum_PI  TsampFilterVariant=InternalTs  TsampNgainVariant=Passthrough  TsampIntegralVariant=Passthrough  ExternalSaturationOutDataTypeStr=Inherit: Same as second input
  Saturation : Saturate  UpperLimit=30000  LowerLimit=-30000
  Sum4 : Sum  Inputs=|+-
  dT1 : Outport
  wires:
  Sum4/1 -> PID Controller/1
  lamda1/1 -> Sum4/2
  PID Controller/1 -> Saturation/1  "dT1"
  p/1 -> PID Controller/2
  i/1 -> PID Controller/3
  Constant/1 -> Sum4/1
  Saturation/1 -> dT1/1

== system tractor_mu1109/驱动防滑模块/Subsystem1 ==
  lamda2 : Inport
  p : Inport  Port=2
  i : Inport  Port=3
  b : Inport  Port=4
  Constant : Constant  Value=0.2
  PID Controller : slpidlib/PID Controller  Controller=PI  Form=Parallel  TimeDomain=Discrete-time  UseExternalTs=off  SampleTime=-1  IntegratorMethod=Forward Euler  FilterMethod=Forward Euler  ControllerParametersSource=external  P=5000  I=3000  UseKiTs=off  D=0  N=100  UseFilter=on  TunerSelectOption=Transfer Function Based (PID Tuner App)  InitialConditionSource=internal  InitialConditionForIntegrator=0  InitialConditionForFilter=0  DifferentiatorICPrevScaledInput=0  ExternalReset=none  TrackingMode=off  Kt=1  LimitOutput=on  SatLimitsSource=internal  UpperSaturationLimit=0  LowerSaturationLimit=-30000  LinearizeAsGain=on  AntiWindupMode=clamping  Kb=1  LimitIntegrator=off  UpperIntegratorSaturationLimit=inf  LowerIntegratorSaturationLimit=-inf  POutMin=[]  POutMax=[]  IOutMin=[]  IOutMax=[]  DOutMin=[]  DOutMax=[]  NOutMin=[]  NOutMax=[]  SumOutMin=[]  SumOutMax=[]  SaturationOutMin=[]  SaturationOutMax=[]  PParamMin=[]  PParamMax=[]  IParamMin=[]  IParamMax=[]  DParamMin=[]  DParamMax=[]  NParamMin=[]  NParamMax=[]  KbParamMin=[]  KbParamMax=[]  KtParamMin=[]  KtParamMax=[]  KbOutMin=[]  KbOutMax=[]  KtOutMin=[]  KtOutMax=[]  IntegratorOutMin=[]  IntegratorOutMax=[]  FilterOutMin=[]  FilterOutMax=[]  SumI1OutMin=[]  SumI1OutMax=[]  SumI2OutMin=[]  SumI2OutMax=[]  SumI3OutMin=[]  SumI3OutMax=[]  SumI4OutMin=[]  SumI4OutMax=[]  SumDOutMin=[]  SumDOutMax=[]  DifferentiatorOutMin=[]  DifferentiatorOutMax=[]  FilterDiffOutCoefMin=[]  FilterDiffOutCoefMax=[]  ReciprocalOutMin=[]  ReciprocalOutMax=[]  SumDenOutMin=[]  SumDenOutMax=[]  SumNumOutMin=[]  SumNumOutMax=[]  DivideOutMin=[]  DivideOutMax=[]  UdiffTsProdOutMin=[]  UdiffTsProdOutMax=[]  NTsProdOutMin=[]  NTsProdOutMax=[]  UintegralTsProdOutMin=[]  UintegralTsProdOutMax=[]  UngainTsProdOutMin=[]  UngainTsProdOutMax=[]  ClampingZeroOutDataTypeStr=Inherit: Inherit via back propagation  ClampingZeroOutMin=[]  ClampingZeroOutMax=[]  FilterDenConstantOutDataTypeStr=Inherit: Inherit via back propagation  FilterDenConstantOutMin=[]  FilterDenConstantOutMax=[]  PCopyOutDataTypeStr=Inherit: Inherit via back propagation  PCopyOutMin=[]  PCopyOutMax=[]  NCopyOutDataTypeStr=Inherit: Inherit via back propagation  NCopyOutMin=[]  NCopyOutMax=[]  IntegratorContinuousStateAttributes=''  IntegratorStateMustResolveToSignalObject=off  IntegratorRTWStateStorageClass=Auto  FilterContinuousStateAttributes=''  FilterStateMustResolveToSignalObject=off  FilterRTWStateStorageClass=Auto  ParallelPVariant=ExternalParameters  IdealPVariant=Disabled  IVariant=ExternalParameters  DVariant=Disabled  IntegratorVariant=Discrete  SatVariant=Enabled  AWVariant=DiscClampingParallel  PCopyVariant=Disabled  TRVariant=Disabled  FdbkBlocksVariant=Forward  IdealPFdbkVariant=Disabled  SatFdbkVariant=Disabled  DerivativeFilterVariant=Disabled  NVariant=Disabled  NCopyVariant=Disabled_SignalSpec  FilterICVariant=Disabled  IntegratorICVariant=InternalICs  ExternalResetVariant=Disabled  TRSumVariant=Passthrough  SumFdbkVariant=Disabled  SumVariant=Sum_PI  TsampFilterVariant=InternalTs  TsampNgainVariant=Passthrough  TsampIntegralVariant=Passthrough  ExternalSaturationOutDataTypeStr=Inherit: Same as second input
  Saturation : Saturate  UpperLimit=30000  LowerLimit=-99999
  Sum4 : Sum  Inputs=|+-
  dT1 : Outport
  wires:
  i/1 -> PID Controller/3
  p/1 -> PID Controller/2
  PID Controller/1 -> Saturation/1  "dT1"
  lamda2/1 -> Sum4/2
  Sum4/1 -> PID Controller/1
  Saturation/1 -> dT1/1
  Constant/1 -> Sum4/1

== system tractor_mu1109/驱动防滑模块/Subsystem2 ==
  lamda3 : Inport
  p : Inport  Port=2
  i : Inport  Port=3
  b : Inport  Port=4
  Constant : Constant  Value=0.2
  PID Controller : slpidlib/PID Controller  Controller=PI  Form=Parallel  TimeDomain=Discrete-time  UseExternalTs=off  SampleTime=-1  IntegratorMethod=Forward Euler  FilterMethod=Forward Euler  ControllerParametersSource=external  P=5000  I=3000  UseKiTs=off  D=0  N=100  UseFilter=on  TunerSelectOption=Transfer Function Based (PID Tuner App)  InitialConditionSource=internal  InitialConditionForIntegrator=0  InitialConditionForFilter=0  DifferentiatorICPrevScaledInput=0  ExternalReset=none  TrackingMode=off  Kt=1  LimitOutput=on  SatLimitsSource=internal  UpperSaturationLimit=0  LowerSaturationLimit=-50000  LinearizeAsGain=on  AntiWindupMode=clamping  Kb=1  LimitIntegrator=off  UpperIntegratorSaturationLimit=inf  LowerIntegratorSaturationLimit=-inf  POutMin=[]  POutMax=[]  IOutMin=[]  IOutMax=[]  DOutMin=[]  DOutMax=[]  NOutMin=[]  NOutMax=[]  SumOutMin=[]  SumOutMax=[]  SaturationOutMin=[]  SaturationOutMax=[]  PParamMin=[]  PParamMax=[]  IParamMin=[]  IParamMax=[]  DParamMin=[]  DParamMax=[]  NParamMin=[]  NParamMax=[]  KbParamMin=[]  KbParamMax=[]  KtParamMin=[]  KtParamMax=[]  KbOutMin=[]  KbOutMax=[]  KtOutMin=[]  KtOutMax=[]  IntegratorOutMin=[]  IntegratorOutMax=[]  FilterOutMin=[]  FilterOutMax=[]  SumI1OutMin=[]  SumI1OutMax=[]  SumI2OutMin=[]  SumI2OutMax=[]  SumI3OutMin=[]  SumI3OutMax=[]  SumI4OutMin=[]  SumI4OutMax=[]  SumDOutMin=[]  SumDOutMax=[]  DifferentiatorOutMin=[]  DifferentiatorOutMax=[]  FilterDiffOutCoefMin=[]  FilterDiffOutCoefMax=[]  ReciprocalOutMin=[]  ReciprocalOutMax=[]  SumDenOutMin=[]  SumDenOutMax=[]  SumNumOutMin=[]  SumNumOutMax=[]  DivideOutMin=[]  DivideOutMax=[]  UdiffTsProdOutMin=[]  UdiffTsProdOutMax=[]  NTsProdOutMin=[]  NTsProdOutMax=[]  UintegralTsProdOutMin=[]  UintegralTsProdOutMax=[]  UngainTsProdOutMin=[]  UngainTsProdOutMax=[]  ClampingZeroOutDataTypeStr=Inherit: Inherit via back propagation  ClampingZeroOutMin=[]  ClampingZeroOutMax=[]  FilterDenConstantOutDataTypeStr=Inherit: Inherit via back propagation  FilterDenConstantOutMin=[]  FilterDenConstantOutMax=[]  PCopyOutDataTypeStr=Inherit: Inherit via back propagation  PCopyOutMin=[]  PCopyOutMax=[]  NCopyOutDataTypeStr=Inherit: Inherit via back propagation  NCopyOutMin=[]  NCopyOutMax=[]  IntegratorContinuousStateAttributes=''  IntegratorStateMustResolveToSignalObject=off  IntegratorRTWStateStorageClass=Auto  FilterContinuousStateAttributes=''  FilterStateMustResolveToSignalObject=off  FilterRTWStateStorageClass=Auto  ParallelPVariant=ExternalParameters  IdealPVariant=Disabled  IVariant=ExternalParameters  DVariant=Disabled  IntegratorVariant=Discrete  SatVariant=Enabled  AWVariant=DiscClampingParallel  PCopyVariant=Disabled  TRVariant=Disabled  FdbkBlocksVariant=Forward  IdealPFdbkVariant=Disabled  SatFdbkVariant=Disabled  DerivativeFilterVariant=Disabled  NVariant=Disabled  NCopyVariant=Disabled_SignalSpec  FilterICVariant=Disabled  IntegratorICVariant=InternalICs  ExternalResetVariant=Disabled  TRSumVariant=Passthrough  SumFdbkVariant=Disabled  SumVariant=Sum_PI  TsampFilterVariant=InternalTs  TsampNgainVariant=Passthrough  TsampIntegralVariant=Passthrough  ExternalSaturationOutDataTypeStr=Inherit: Same as second input
  Saturation : Saturate  UpperLimit=30000  LowerLimit=-99999
  Sum4 : Sum  Inputs=|+-
  dT1 : Outport
  wires:
  Sum4/1 -> PID Controller/1
  lamda3/1 -> Sum4/2
  PID Controller/1 -> Saturation/1  "dT1"
  p/1 -> PID Controller/2
  i/1 -> PID Controller/3
  Saturation/1 -> dT1/1
  Constant/1 -> Sum4/1

== system tractor_mu1109/驱动防滑模块/Subsystem3 ==
  lamda4 : Inport
  p : Inport  Port=2
  i : Inport  Port=3
  b : Inport  Port=4
  Constant : Constant  Value=0.2
  PID Controller : slpidlib/PID Controller  Controller=PI  Form=Parallel  TimeDomain=Discrete-time  UseExternalTs=off  SampleTime=-1  IntegratorMethod=Forward Euler  FilterMethod=Forward Euler  ControllerParametersSource=external  P=5000  I=3000  UseKiTs=off  D=0  N=100  UseFilter=on  TunerSelectOption=Transfer Function Based (PID Tuner App)  InitialConditionSource=internal  InitialConditionForIntegrator=0  InitialConditionForFilter=0  DifferentiatorICPrevScaledInput=0  ExternalReset=none  TrackingMode=off  Kt=1  LimitOutput=on  SatLimitsSource=internal  UpperSaturationLimit=0  LowerSaturationLimit=-50000  LinearizeAsGain=on  AntiWindupMode=clamping  Kb=1  LimitIntegrator=off  UpperIntegratorSaturationLimit=inf  LowerIntegratorSaturationLimit=-inf  POutMin=[]  POutMax=[]  IOutMin=[]  IOutMax=[]  DOutMin=[]  DOutMax=[]  NOutMin=[]  NOutMax=[]  SumOutMin=[]  SumOutMax=[]  SaturationOutMin=[]  SaturationOutMax=[]  PParamMin=[]  PParamMax=[]  IParamMin=[]  IParamMax=[]  DParamMin=[]  DParamMax=[]  NParamMin=[]  NParamMax=[]  KbParamMin=[]  KbParamMax=[]  KtParamMin=[]  KtParamMax=[]  KbOutMin=[]  KbOutMax=[]  KtOutMin=[]  KtOutMax=[]  IntegratorOutMin=[]  IntegratorOutMax=[]  FilterOutMin=[]  FilterOutMax=[]  SumI1OutMin=[]  SumI1OutMax=[]  SumI2OutMin=[]  SumI2OutMax=[]  SumI3OutMin=[]  SumI3OutMax=[]  SumI4OutMin=[]  SumI4OutMax=[]  SumDOutMin=[]  SumDOutMax=[]  DifferentiatorOutMin=[]  DifferentiatorOutMax=[]  FilterDiffOutCoefMin=[]  FilterDiffOutCoefMax=[]  ReciprocalOutMin=[]  ReciprocalOutMax=[]  SumDenOutMin=[]  SumDenOutMax=[]  SumNumOutMin=[]  SumNumOutMax=[]  DivideOutMin=[]  DivideOutMax=[]  UdiffTsProdOutMin=[]  UdiffTsProdOutMax=[]  NTsProdOutMin=[]  NTsProdOutMax=[]  UintegralTsProdOutMin=[]  UintegralTsProdOutMax=[]  UngainTsProdOutMin=[]  UngainTsProdOutMax=[]  ClampingZeroOutDataTypeStr=Inherit: Inherit via back propagation  ClampingZeroOutMin=[]  ClampingZeroOutMax=[]  FilterDenConstantOutDataTypeStr=Inherit: Inherit via back propagation  FilterDenConstantOutMin=[]  FilterDenConstantOutMax=[]  PCopyOutDataTypeStr=Inherit: Inherit via back propagation  PCopyOutMin=[]  PCopyOutMax=[]  NCopyOutDataTypeStr=Inherit: Inherit via back propagation  NCopyOutMin=[]  NCopyOutMax=[]  IntegratorContinuousStateAttributes=''  IntegratorStateMustResolveToSignalObject=off  IntegratorRTWStateStorageClass=Auto  FilterContinuousStateAttributes=''  FilterStateMustResolveToSignalObject=off  FilterRTWStateStorageClass=Auto  ParallelPVariant=ExternalParameters  IdealPVariant=Disabled  IVariant=ExternalParameters  DVariant=Disabled  IntegratorVariant=Discrete  SatVariant=Enabled  AWVariant=DiscClampingParallel  PCopyVariant=Disabled  TRVariant=Disabled  FdbkBlocksVariant=Forward  IdealPFdbkVariant=Disabled  SatFdbkVariant=Disabled  DerivativeFilterVariant=Disabled  NVariant=Disabled  NCopyVariant=Disabled_SignalSpec  FilterICVariant=Disabled  IntegratorICVariant=InternalICs  ExternalResetVariant=Disabled  TRSumVariant=Passthrough  SumFdbkVariant=Disabled  SumVariant=Sum_PI  TsampFilterVariant=InternalTs  TsampNgainVariant=Passthrough  TsampIntegralVariant=Passthrough  ExternalSaturationOutDataTypeStr=Inherit: Same as second input
  Saturation : Saturate  UpperLimit=30000  LowerLimit=-99999
  Sum4 : Sum  Inputs=|+-
  dT1 : Outport
  wires:
  i/1 -> PID Controller/3
  p/1 -> PID Controller/2
  PID Controller/1 -> Saturation/1  "dT1"
  lamda4/1 -> Sum4/2
  Sum4/1 -> PID Controller/1
  Saturation/1 -> dT1/1
  Constant/1 -> Sum4/1
